simulink model "sparrow_albatros_spec_withgpio_bram"  (R2021a)
settings: Solver=VariableStepDiscrete  StartTime=0.0  StopTime=200000  RelTol=1e-3
undefined symbols (not defined in the file): pfb_coeff_gen_calc
libraries: xbsIndex_r4 x5629, casper_library_misc x33, casper_library_delays x28, xps_library x10, simulink x8, xbsReplacements_r4 x2
(part 25 of 85)

== system sparrow_albatros_spec_withgpio_bram/tvg1/enable ==
  sim_1 : Inport
  convert1_1 : DataTypeConversion  OutDataTypeStr=fixdt('ufix1_En0')  LockScale=on
  convert2_1 : DataTypeConversion  OutDataTypeStr=fixdt('ufix1_En0')  ConvertRealWorld=Stored Integer (SI)  LockScale=on
  gain_1 : Gain  OutDataTypeStr=fixdt('ufix32_En0')
  io_delay : xbsIndex_r4/Delay  rst=off  infoeditControl=Selection of Reset will increase slice count due to use of real FFs and instead of SRLs  en=off  latency=0  reg_retiming=on  dbl_ovrd=off  block_type=delay
  reint1 : xbsIndex_r4/Reinterpret  force_arith_type=on  arith_type=Unsigned  force_bin_pt=on  bin_pt=0  block_type=reinterpret
  slice_reg : xbsIndex_r4/Slice  nbits=1  boolean_output=off  mode=Lower Bit Location + Width  bit1=0  base1=MSB of Input  bit0=0  base0=LSB of Input  dbl_ovrd=off  block_type=slice
  sparrow_albatros_spec_withgpio_bram_tvg1_enable_user_data_out : xbsIndex_r4/Gateway In  gui_display_data_type=Fixed-point  arith_type=Unsigned  n_bits=32  bin_pt=0  preci_type=Single  exp_width=8  frac_width=24  rows=1  columns=1  quantization="Round  (unbiased: +/- Inf)"  overflow=Saturate  period=1  UseAsADC=off  ADCChannel='1'  interface=None  automatic_assignment=on  address_offset=hex2dec('00')  intf_name=''  intf_description=''  default_value=0  timing_constraint=None  locs_specified=off  LOCs={}  io_standard={}  inherit_from_input=off  hdl_port=on  dbl_ovrd=off  block_type=gatewayin
  in_reg : Outport  VectorParamsAs1DForOutWhenUnconnected=off
  wires:
  sparrow_albatros_spec_withgpio_bram_tvg1_enable_user_data_out/1 -> io_delay/1
  sim_1/1 -> convert1_1/1
  convert1_1/1 -> convert2_1/1
  convert2_1/1 -> gain_1/1
  gain_1/1 -> sparrow_albatros_spec_withgpio_bram_tvg1_enable_user_data_out/1
  io_delay/1 -> slice_reg/1
  slice_reg/1 -> reint1/1
  reint1/1 -> in_reg/1

== system sparrow_albatros_spec_withgpio_bram/tvg16bit/bus_expand1 ==
  bus_in : Inport
  reinterpret1 : xbsIndex_r4/Reinterpret  force_arith_type=on  arith_type=Unsigned  force_bin_pt=on  bin_pt=0  block_type=reinterpret
  reinterpret2 : xbsIndex_r4/Reinterpret  force_arith_type=on  arith_type=Unsigned  force_bin_pt=on  bin_pt=0  block_type=reinterpret
  slice1 : xbsIndex_r4/Slice  nbits=8  boolean_output=off  mode=Upper Bit Location + Width  bit1=-8  base1=MSB of Input  bit0=0  base0=LSB of Input  dbl_ovrd=off  block_type=slice
  slice2 : xbsIndex_r4/Slice  nbits=8  boolean_output=off  mode=Upper Bit Location + Width  bit1=0  base1=MSB of Input  bit0=0  base0=LSB of Input  dbl_ovrd=off  block_type=slice
  msb_out2 : Outport  VectorParamsAs1DForOutWhenUnconnected=off
  lsb_out1 : Outport  Port=2  VectorParamsAs1DForOutWhenUnconnected=off
  wires:
  bus_in/1 -> slice2/1, slice1/1
  slice2/1 -> reinterpret2/1
  reinterpret2/1 -> msb_out2/1
  slice1/1 -> reinterpret1/1
  reinterpret1/1 -> lsb_out1/1

== system sparrow_albatros_spec_withgpio_bram/tvg16bit/data ==
  addr : Inport
  data_in : Inport  Port=2
  we : Inport  Port=3
  Terminator : Terminator
  Terminator1 : Terminator
  Terminator2 : Terminator
  calc_add : Subsystem  mask{data_width=32, addr_width=11, sample_rate=sample_rate}
      mask prompts: data_width "data width"; addr_width "address width"; sample_rate "sample rate"
  convert_addr : xbsIndex_r4/Convert  gui_display_data_type=Fixed-point  arith_type=Unsigned  n_bits=addr_width  bin_pt=0  float_type=Single  exp_bits=8  fraction_bits=24  quantization=Truncate  overflow=Wrap  en=off  latency=0  pipeline=off  dbl_ovrd=off  block_type=convert
      settings: xl_area=[0, 0, 0, 0, 0, 0, 0]
  convert_din1 : xbsIndex_r4/Convert  gui_display_data_type=Fixed-point  arith_type=Unsigned  n_bits=32  bin_pt=0  float_type=Single  exp_bits=8  fraction_bits=24  quantization=Truncate  overflow=Wrap  en=off  latency=0  pipeline=off  dbl_ovrd=off  block_type=convert
      settings: xl_area=[0, 0, 0, 0, 0, 0, 0]
  convert_we : xbsIndex_r4/Convert  gui_display_data_type=Fixed-point  arith_type=Unsigned  n_bits=1  bin_pt=0  float_type=Single  exp_bits=8  fraction_bits=24  quantization=Truncate  overflow=Wrap  en=off  latency=0  pipeline=off  dbl_ovrd=off  block_type=convert
      settings: xl_area=[0, 0, 0, 0, 0, 0, 0]
  munge_in : Subsystem  AncestorBlock=casper_library_flow_control/munge  mask(munge){divisions=1, div_size=32, order=[0], arith_type_out=Unsigned, bin_pt_out=0}
      mask prompts: divisions "Number of divisions"; div_size "Division size (bits)"; order "Division packing order"; arith_type_out "Output arithmetic type"; bin_pt_out "Output binary point"
      mask help: Splits an input bus into the specified number of divisions and then recombines them in the order specified (most significant division = 0,least = number divisions-1)
      mask init:
      | munge_init(gcb, ...
      |     'divisions', divisions, ...
      |     'div_size', div_size, ...
      |     'order', order, ...
      |     'arith_type_out', arith_type_out, ...
      |     'bin_pt_out', bin_pt_out);
      settings: AttributesFormatString=|
      | split:32
      | join:0
      | Unsigned [32,0]
      mask TypeOptions arith_type_out: Unsigned | Signed  (2's comp) | Floating-point
  munge_out : Subsystem  AncestorBlock=casper_library_flow_control/munge  mask(munge){divisions=1, div_size=32, order=[0], arith_type_out=Unsigned, bin_pt_out=0}
      mask prompts: divisions "Number of divisions"; div_size "Division size (bits)"; order "Division packing order"; arith_type_out "Output arithmetic type"; bin_pt_out "Output binary point"
      mask help: Splits an input bus into the specified number of divisions and then recombines them in the order specified (most significant division = 0,least = number divisions-1)
      mask init:
      | munge_init(gcb, ...
      |     'divisions', divisions, ...
      |     'div_size', div_size, ...
      |     'order', order, ...
      |     'arith_type_out', arith_type_out, ...
      |     'bin_pt_out', bin_pt_out);
      settings: AttributesFormatString=|
      | split:32
      | join:0
      | Unsigned [32,0]
      mask TypeOptions arith_type_out: Unsigned | Signed  (2's comp) | Floating-point
  sim_mem : Subsystem  mask{arith_type=Unsigned, addr_width=11, data_width=32, data_bin_pt=0, init_vals=[0    257    514    771   1028   1285   1542   1799   2056   2313   2570   2827   3084   3341   3598   3855   4112   4369   4626   4883   5140   5397   5654   5911   6168   6425   6682   6939   7196   7453   7710   7967   8224   8481   8738   8995   9252   9509   9766  10023  10280  10537  10794  11051  11308  11565  11822  12079  12336  12593  12850  13107  13364  13621  13878  14135  14392  14649  14906  15163  15420  15677  15934  16191  16448  16705  16962  17219  17476  17733  17990  18247  18504  18761  19018  19275  19532  19789  20046  20303  20560  20817  21074  21331  21588  21845  22102  22359  22616  22873  23130  23387  23644  23901  24158  24415  24672  24929  25186  25443  25700  25957  26214  26471  26728  26985  27242  27499  27756  28013  28270  28527  28784  29041  29298  29555  29812  30069  30326  30583  30840  31097  31354  31611  31868  32125  32382  32639  32896  33153  33410  33667  33924  34181  34438  34695  34952  35209  35466  35723  35980  36237  36494  36751  37008  37265  37522  37779  38036  38293  38550  38807  39064  39321  39578  39835  40092  40349  40606  40863  41120  41377  41634  41891  42148  42405  42662  42919  43176  43433  43690  43947  44204  44461  44718  44975  45232  45489  45746  46003  46260  46517  46774  47031  47288  47545  47802  48059  48316  48573  48830  49087  49344  49601  49858  50115  50372  50629  50886  51143  51400  51657  51914  52171  52428  52685  52942  53199  53456  53713  53970  54227  54484  54741  54998  55255  55512  55769  56026  56283  56540  56797  57054  57311  57568  57825  58082  58339  58596  58853  59110  59367  59624  59881  60138  60395  60652  60909  61166  61423  61680  61937  62194  62451  62708  62965  63222  63479  63736  63993  64250  64507  64764  65021  65278  65535      0    257    514    771   1028   1285   1542   1799   2056   2313   2570   2827   3084   3341   3598   3855   4112   4369   4626   4883   5140   5397   5654   5911   6168   6425   6682   6939   7196   7453   7710   7967   8224   8481   8738   8995   9252   9509   9766  10023  10280  10537  10794  11051  11308  11565  11822  12079  12336  12593  12850  13107  13364  13621  13878  14135  14392  14649  14906  15163  15420  15677  15934  16191  16448  16705  16962  17219  17476  17733  17990  18247  18504  18761  19018  19275  19532  19789  20046  20303  20560  20817  21074  21331  21588  21845  22102  22359  22616  22873  23130  23387  23644  23901  24158  24415  24672  24929  25186  25443  25700  25957  26214  26471  26728  26985  27242  27499  27756  28013  28270  28527  28784  29041  29298  29555  29812  30069  30326  30583  30840  31097  31354  31611  31868  32125  32382  32639  32896  33153  33410  33667  33924  34181  34438  34695  34952  35209  35466  35723  35980  36237  36494  36751  37008  37265  37522  37779  38036  38293  38550  38807  39064  39321  39578  39835  40092  40349  40606  40863  41120  41377  41634  41891  42148  42405  42662  42919  43176  43433  43690  43947  44204  44461  44718  44975  45232  45489  45746  46003  46260  46517  46774  47031  47288  47545  47802  48059  48316  48573  48830  49087  49344  49601  49858  50115  50372  50629  50886  51143  51400  51657  51914  52171  52428  52685  52942  53199  53456  53713  53970  54227  54484  54741  54998  55255  55512  55769  56026  56283  56540  56797  57054  57311  57568  57825  58082  58339  58596  58853  59110  59367  59624  59881  60138  60395  60652  60909  61166  61423  61680  61937  62194  62451  62708  62965  63222  63479  63736  63993  64250  64507  64764  65021  65278  65535      0    257    514    771   1028   1285   1542   1799   2056   2313   2570   2827   3084   3341   3598   3855   4112   4369   4626   4883   5140   5397   5654   5911   6168   6425   6682   6939   7196   7453   7710   7967   8224   8481   8738   8995   9252   9509   9766  10023  10280  10537  10794  11051  11308  11565  11822  12079  12336  12593  12850  13107  13364  13621  13878  14135  14392  14649  14906  15163 ...(+10332 chars)], sample_rate=1, csp_latency=1}
      mask prompts: arith_type "Output Data Type"; addr_width "Address width"; data_width "Data width"; data_bin_pt "Data Binary Point"; init_vals "Initial values"; sample_rate "Sample rate"; csp_latency "Latency"
      mask init:
      | % set_param([gcb, '/data_to_xilinx'], 'arith_type', arith_type)
      | % set_param([gcb, '/data_to_xilinx'], 'n_bits', get_param(gcb, 'data_width'))
      mask TypeOptions arith_type: Unsigned | Signed  (2's comp)
      mask TypeOptions data_width: 8 | 16 | 32 | 64 | 128
  sparrow_albatros_spec_withgpio_bram_tvg16bit_data_addr : xbsIndex_r4/Gateway Out  inherit_from_input=off  hdl_port=on  rows=1  columns=1  UseAsDAC=off  DACChannel='1'  interface=None  automatic_assignment=on  address_offset=hex2dec('00')  intf_name=''  intf_description=''  timing_constraint=None  locs_specified=off  LOCs={'A5','B9','A9','C1','A3','G6','E9','A6','A7','A8','B8','B1','B3','D9','B5','B4','B6','C2'}  io_standard={}  block_type=gatewayout
      settings: infoedit="Gateway out block.  Converts Xilinx fixed point inputs into ouputs of type Simulink integer, double, or fixed point.<P><P>Hardware notes:  In hardware these blocks become top level output ports or are discarded, depending on how they are configured."  sginterface={'Nallatech'=>{'xdspkit'=>{'non_memory_mapped_port'=>'uprev_Shared_BRAM_addr'}},'Xilinx'=>{'jtaghwcosim'=>{'non_memory_mapped_port'=>'uprev_Shared_BRAM_addr'},'xdspkit'=>{'non_memory_mapped_port'=>'uprev_Shared_BRAM_addr'}}}  xl_area=[0, 0, 0, 0, 0, 0, 0]
  sparrow_albatros_spec_withgpio_bram_tvg16bit_data_data_in : xbsIndex_r4/Gateway Out  inherit_from_input=off  hdl_port=on  rows=1  columns=1  UseAsDAC=off  DACChannel='1'  interface=None  automatic_assignment=on  address_offset=hex2dec('00')  intf_name=''  intf_description=''  timing_constraint=None  locs_specified=off  LOCs={'B21','B22','A22','B23','B19','C19','A20','A21','A23','B24','A24','A25','E18','D18','C18','B18'}  io_standard={}  block_type=gatewayout
      settings: infoedit="Gateway out block.  Converts Xilinx fixed point inputs into ouputs of type Simulink integer, double, or fixed point.<P><P>Hardware notes:  In hardware these blocks become top level output ports or are discarded, depending on how they are configured."  sginterface={'Nallatech'=>{'xdspkit'=>{'non_memory_mapped_port'=>'uprev_Shared_BRAM_data_in'}},'Xilinx'=>{'jtaghwcosim'=>{'non_memory_mapped_port'=>'uprev_Shared_BRAM_data_in'},'xdspkit'=>{'non_memory_mapped_port'=>'uprev_Shared_BRAM_data_in'}}}  xl_area=[0, 0, 0, 0, 0, 0, 0]
  sparrow_albatros_spec_withgpio_bram_tvg16bit_data_data_out : xbsIndex_r4/Gateway In  gui_display_data_type=Fixed-point  arith_type=Unsigned  n_bits=32  bin_pt=0  preci_type=Single  exp_width=8  frac_width=24  rows=1  columns=1  quantization=Truncate  overflow=Wrap  period=sample_rate  UseAsADC=off  ADCChannel='1'  interface=None  automatic_assignment=on  address_offset=hex2dec('00')  intf_name=''  intf_description=''  default_value=0  timing_constraint=None  locs_specified=off  LOCs={}  io_standard={}  inherit_from_input=off  hdl_port=on  dbl_ovrd=off  block_type=gatewayin
      settings: xl_area=[0, 0, 0, 0, 0, 0, 0]
  sparrow_albatros_spec_withgpio_bram_tvg16bit_data_we : xbsIndex_r4/Gateway Out  inherit_from_input=off  hdl_port=on  rows=1  columns=1  UseAsDAC=off  DACChannel='1'  interface=None  automatic_assignment=on  address_offset=hex2dec('00')  intf_name=''  intf_description=''  timing_constraint=None  locs_specified=off  LOCs={'A14'}  io_standard={}  block_type=gatewayout
      settings: infoedit="Gateway out block.  Converts Xilinx fixed point inputs into ouputs of type Simulink integer, double, or fixed point.<P><P>Hardware notes:  In hardware these blocks become top level output ports or are discarded, depending on how they are configured."  xl_area=[0, 0, 0, 0, 0, 0, 0]
  data_out : Outport  VectorParamsAs1DForOutWhenUnconnected=off
  wires:
  munge_out/1(dout) -> data_out/1
  sim_mem/1(data_out) -> sparrow_albatros_spec_withgpio_bram_tvg16bit_data_data_out/1
  sparrow_albatros_spec_withgpio_bram_tvg16bit_data_data_out/1 -> munge_out/1(din)
  convert_addr/1 -> sparrow_albatros_spec_withgpio_bram_tvg16bit_data_addr/1
  convert_din1/1 -> sparrow_albatros_spec_withgpio_bram_tvg16bit_data_data_in/1
  data_in/1 -> munge_in/1(din)
  calc_add/1(out) -> sim_mem/1(addr), convert_addr/1
  sparrow_albatros_spec_withgpio_bram_tvg16bit_data_we/1 -> Terminator2/1
  sparrow_albatros_spec_withgpio_bram_tvg16bit_data_data_in/1 -> Terminator1/1
  sparrow_albatros_spec_withgpio_bram_tvg16bit_data_addr/1 -> Terminator/1
  convert_we/1 -> sparrow_albatros_spec_withgpio_bram_tvg16bit_data_we/1
  addr/1 -> calc_add/1(in)
  we/1 -> sim_mem/3(we), convert_we/1
  munge_in/1(dout) -> sim_mem/2(data), convert_din1/1

== system sparrow_albatros_spec_withgpio_bram/tvg16bit/enable ==
  sim_1 : Inport
  convert1_1 : DataTypeConversion  OutDataTypeStr=fixdt('ufix1_En0')  LockScale=on
  convert2_1 : DataTypeConversion  OutDataTypeStr=fixdt('ufix1_En0')  ConvertRealWorld=Stored Integer (SI)  LockScale=on
  gain_1 : Gain  OutDataTypeStr=fixdt('ufix32_En0')
  io_delay : xbsIndex_r4/Delay  rst=off  infoeditControl=Selection of Reset will increase slice count due to use of real FFs and instead of SRLs  en=off  latency=0  reg_retiming=on  dbl_ovrd=off  block_type=delay
  reint1 : xbsIndex_r4/Reinterpret  force_arith_type=on  arith_type=Unsigned  force_bin_pt=on  bin_pt=0  block_type=reinterpret
  slice_reg : xbsIndex_r4/Slice  nbits=1  boolean_output=off  mode=Lower Bit Location + Width  bit1=0  base1=MSB of Input  bit0=0  base0=LSB of Input  dbl_ovrd=off  block_type=slice
  sparrow_albatros_spec_withgpio_bram_tvg16bit_enable_user_data_out : xbsIndex_r4/Gateway In  gui_display_data_type=Fixed-point  arith_type=Unsigned  n_bits=32  bin_pt=0  preci_type=Single  exp_width=8  frac_width=24  rows=1  columns=1  quantization="Round  (unbiased: +/- Inf)"  overflow=Saturate  period=1  UseAsADC=off  ADCChannel='1'  interface=None  automatic_assignment=on  address_offset=hex2dec('00')  intf_name=''  intf_description=''  default_value=0  timing_constraint=None  locs_specified=off  LOCs={}  io_standard={}  inherit_from_input=off  hdl_port=on  dbl_ovrd=off  block_type=gatewayin
  in_reg : Outport  VectorParamsAs1DForOutWhenUnconnected=off
  wires:
  sparrow_albatros_spec_withgpio_bram_tvg16bit_enable_user_data_out/1 -> io_delay/1
  sim_1/1 -> convert1_1/1
  convert1_1/1 -> convert2_1/1
  convert2_1/1 -> gain_1/1
  gain_1/1 -> sparrow_albatros_spec_withgpio_bram_tvg16bit_enable_user_data_out/1
  io_delay/1 -> slice_reg/1
  slice_reg/1 -> reint1/1
  reint1/1 -> in_reg/1

== system sparrow_albatros_spec_withgpio_bram/Subsystem/a_replicate/bussify ==
  in1 : Inport
  in2 : Inport  Port=2
  concatenate : xbsIndex_r4/Concat  num_inputs=2  dbl_ovrd=off  block_type=concat
  reinterpret1 : xbsIndex_r4/Reinterpret  force_arith_type=on  arith_type=Unsigned  force_bin_pt=on  bin_pt=0  block_type=reinterpret
      settings: infoedit="Changes signal type without altering the binary representation.   You can changed the signal between signed and unsigned, and relocate the binary point.<br><br>Hardware notes: In hardware this block costs nothing.<br><br>Example:  Suppose the input is 6 bits wide, signed, with 2 fractional bits, and the output is forced to unsigned with 0 fractional bits.  Then an input of -2.0 (1110.00 in binary 2's complement) becomes an output of 56 (111000 in binary)."
  reinterpret2 : xbsIndex_r4/Reinterpret  force_arith_type=on  arith_type=Unsigned  force_bin_pt=on  bin_pt=0  block_type=reinterpret
      settings: infoedit="Changes signal type without altering the binary representation.   You can changed the signal between signed and unsigned, and relocate the binary point.<br><br>Hardware notes: In hardware this block costs nothing.<br><br>Example:  Suppose the input is 6 bits wide, signed, with 2 fractional bits, and the output is forced to unsigned with 0 fractional bits.  Then an input of -2.0 (1110.00 in binary 2's complement) becomes an output of 56 (111000 in binary)."
  bus_out : Outport  VectorParamsAs1DForOutWhenUnconnected=off
  wires:
  concatenate/1 -> bus_out/1
  in1/1 -> reinterpret1/1
  reinterpret1/1 -> concatenate/1
  in2/1 -> reinterpret2/1
  reinterpret2/1 -> concatenate/2

== system sparrow_albatros_spec_withgpio_bram/Subsystem/b_replicate/bussify ==
  in1 : Inport
  in2 : Inport  Port=2
  concatenate : xbsIndex_r4/Concat  num_inputs=2  dbl_ovrd=off  block_type=concat
  reinterpret1 : xbsIndex_r4/Reinterpret  force_arith_type=on  arith_type=Unsigned  force_bin_pt=on  bin_pt=0  block_type=reinterpret
      settings: infoedit="Changes signal type without altering the binary representation.   You can changed the signal between signed and unsigned, and relocate the binary point.<br><br>Hardware notes: In hardware this block costs nothing.<br><br>Example:  Suppose the input is 6 bits wide, signed, with 2 fractional bits, and the output is forced to unsigned with 0 fractional bits.  Then an input of -2.0 (1110.00 in binary 2's complement) becomes an output of 56 (111000 in binary)."
  reinterpret2 : xbsIndex_r4/Reinterpret  force_arith_type=on  arith_type=Unsigned  force_bin_pt=on  bin_pt=0  block_type=reinterpret
      settings: infoedit="Changes signal type without altering the binary representation.   You can changed the signal between signed and unsigned, and relocate the binary point.<br><br>Hardware notes: In hardware this block costs nothing.<br><br>Example:  Suppose the input is 6 bits wide, signed, with 2 fractional bits, and the output is forced to unsigned with 0 fractional bits.  Then an input of -2.0 (1110.00 in binary 2's complement) becomes an output of 56 (111000 in binary)."
  bus_out : Outport  VectorParamsAs1DForOutWhenUnconnected=off
  wires:
  concatenate/1 -> bus_out/1
  in1/1 -> reinterpret1/1
  reinterpret1/1 -> concatenate/1
  in2/1 -> reinterpret2/1
  reinterpret2/1 -> concatenate/2
